simulink model "rfsoc4x2_ospfb_128"  (R2021a)
settings: Solver=VariableStepAuto  StartTime=0.0  StopTime=2048  RelTol=1e-3
undefined symbols (not defined in the file): pfb_coeff_gen_calc
libraries: xbsIndex_r4 x37092, casper_library_delays x737, casper_library_misc x68, xps_library x1
(part 228 of 339)

== system rfsoc4x2_ospfb_128/fft_wideband_real1/fft_direct/butterfly0_0/twiddle/bus_mult ==
  a : Inport
  b : Inport  Port=2
  misci : Inport  Port=3
  a*b_bussify : Subsystem  AncestorBlock=casper_library_flow_control/bus_create  mask(bus_create){inputNum=8}
      mask prompts: inputNum "Number of inputs:"
      mask init:
      | bus_create_init(gcb,...
      |     'inputNum', inputNum);
  a_debus : Subsystem  AncestorBlock=casper_library_flow_control/bus_expand  mask(bus_expand){mode=divisions of arbitrary size, outputNum=2, outputWidth=36, outputBinaryPt=0, outputArithmeticType=0, show_format=on, outputToWorkspace=off, variablePrefix=, outputToModelAsWell=on}
      mask prompts: outputNum "Number of outputs:"; outputWidth "Output width:"; outputBinaryPt "Output binary point position:"; outputArithmeticType "Output arithmetic type (ufix=0, fix=1, bool=2):"; show_format "Print format string?"; outputToWorkspace "Output to workspace?"; variablePrefix "Variable name prefix:"; outputToModelAsWell "Output to model as well?"
      mask help:
      | Expands a 'bus' made using a bus_create or Xilinx
      | concat block.
      | The input will be divided into the specified number
      | of outputs with the specified arithmetic types.
      | Divisions are made from most significant bit.
      mask init: same as rfsoc4x2_ospfb_128/bus_expand1
      settings: AttributesFormatString=1 outputs: uf36.0,
      mask TypeOptions mode: divisions of equal size | divisions of arbitrary size
      mask Callback mode: %bus_expand_callback();
      mask Callback outputWidth: %bus_expand_callback();
      mask Callback outputToWorkspace: %bus_expand_callback();
  b_debus : Subsystem  AncestorBlock=casper_library_flow_control/bus_expand  mask(bus_expand){mode=divisions of arbitrary size, outputNum=2, outputWidth=[36 36 36 36 36 36 36 36], outputBinaryPt=[0 0 0 0 0 0 0 0], outputArithmeticType=[0 0 0 0 0 0 0 0], show_format=on, outputToWorkspace=off, variablePrefix=, outputToModelAsWell=on}
      mask prompts: outputNum "Number of outputs:"; outputWidth "Output width:"; outputBinaryPt "Output binary point position:"; outputArithmeticType "Output arithmetic type (ufix=0, fix=1, bool=2):"; show_format "Print format string?"; outputToWorkspace "Output to workspace?"; variablePrefix "Variable name prefix:"; outputToModelAsWell "Output to model as well?"
      mask help:
      | Expands a 'bus' made using a bus_create or Xilinx
      | concat block.
      | The input will be divided into the specified number
      | of outputs with the specified arithmetic types.
      | Divisions are made from most significant bit.
      mask init: same as rfsoc4x2_ospfb_128/bus_expand1
      settings: AttributesFormatString=8 outputs: uf36.0,uf36.0,uf36.0,uf36.0,uf36.0,uf36.0,uf36.0,uf36.0,
      mask TypeOptions mode: divisions of equal size | divisions of arbitrary size
      mask Callback mode: %bus_expand_callback();
      mask Callback outputWidth: %bus_expand_callback();
      mask Callback outputToWorkspace: %bus_expand_callback();
  dmisc : xbsIndex_r4/Delay  rst=off  infoeditControl=Selection of Reset will increase slice count due to use of real FFs and instead of SRLs  en=off  latency=mult_latency+add_latency+conv_latency+fan_latency  reg_retiming=on  dbl_ovrd=off  block_type=delay
  mult1 : Subsystem  AncestorBlock=casper_library_multipliers/cmult  mask(cmult){n_bits_a=18, bin_pt_a=17, n_bits_b=18, bin_pt_b=17, n_bits_ab=37, bin_pt_ab=34, quantization=Truncate, overflow=Wrap, conjugated=off, async=off, pipelined_enable=on, floating_point=off, float_type=single, exp_width=8, frac_width=24, in_latency=0, mult_latency=3, add_latency=1, conv_latency=0, pipeline_cmult_en=off, pipeline_latency=0, multiplier_implementation=behavioral HDL}
      mask prompts: n_bits_a "Number of Bits 'a'"; bin_pt_a "Binary Point 'a'"; n_bits_b "Number of Bits 'b'"; bin_pt_b "Binary Point 'b'"; n_bits_ab "Number of Bits 'ab'"; bin_pt_ab "Binary Point 'ab'"; conjugated "Conjugate"; async "asynchronous operation"; pipelined_enable "enable pipeline"; floating_point "floating point"; float_type "float type"; exp_width "exponent width"; frac_width "fraction width"; in_latency "Input latency"; mult_latency "Multiplier Latency"; add_latency "Adder Latency"; conv_latency "Convert latency"; pipeline_cmult_en "Pipeline cmult enable"; pipeline_latency "Pipeline latency"; multiplier_implementation "Multiplier implementation"
      mask help:
      | Multiplies two complex numbers using 4 multipliers and 2 adders.
      | Conjugation is optional.
      mask init: same as rfsoc4x2_ospfb_128/fft2/fft_direct/butterfly0_0/twiddle/bus_mult/mult1
      settings: AttributesFormatString=|
      | 18_17 * 18_17 ==> 37_34
      | Truncate, Wrap
      | Latency=0
      mask TypeOptions quantization: Truncate | Round  (unbiased: +/- Inf) | Round  (unbiased: Even Values)
      mask TypeOptions overflow: Wrap | Saturate | Flag as error
      mask Callback floating_point:
      | onoff = get_param(gcb, 'floating_point');
      | if strcmp(onoff,'on')
      |     enable_fixpt = 'off';
      |     set_param_state(gcb, 'float_type', 'on')
      | 
      |     f_type = get_param(gcb, 'float_type');
      |     if strcmp(f_type,'custom')
      |         set_param_state(gcb, 'exp_width', 'on')
      |         set_param_state(gcb, 'frac_width', 'on')
      |     else
      |         set_param_state(gcb, 'exp_width', 'off')
      |         set_param_state(gcb, 'frac_width', 'off')
      |     end
      | 
      | 
      | else
      |     enable_fixpt = 'on';
      |     set_param_state(gcb, 'float_type', 'off')
      |     set_param_state(gcb, 'exp_width', 'off')
      |     set_param_state(gcb, 'frac_width', 'off')
      | end
      | 
      | 
      | set_param_state(gcb, 'n_bits_a', enable_fixpt)
      | set_param_state(gcb, 'bin_pt_a', enable_fixpt)
      | set_param_state(gcb, 'n_bits_b', enable_fixpt)
      | set_param_state(gcb, 'bin_pt_b', enable_fixpt)
      | set_param_state(gcb, 'n_bits_ab', enable_fixpt)
      | set_param_state(gcb, 'bin_pt_ab', enable_fixpt)
      mask TypeOptions float_type: single | custom
      mask Callback float_type:
      | f_type = get_param(gcb, 'float_type');
      | if strcmp(f_type,'custom')
      |     set_param_state(gcb, 'exp_width', 'on')
      |     set_param_state(gcb, 'frac_width', 'on')
      | else
      |     set_param_state(gcb, 'exp_width', 'off')
      |     set_param_state(gcb, 'frac_width', 'off')
      | end
      mask Callback pipeline_cmult_en:
      | pipeline_en = get_param(gcb, 'pipeline_cmult_en');
      | if strcmp(pipeline_en,'on')
      | 
      |     set_param_state(gcb, 'pipeline_latency', 'on')
      | else
      |     set_param_state(gcb, 'pipeline_latency', 'off')
      | end
      mask TypeOptions multiplier_implementation: behavioral HDL | standard core | embedded multiplier core
      mask DialogControl ParameterTabVar0 Prompt: basic
      mask DialogControl ParameterTabVar01 Prompt: latency
      mask DialogControl ParameterTabVar012 Prompt: implementation
  mult2 : Subsystem  AncestorBlock=casper_library_multipliers/cmult  mask(cmult){n_bits_a=18, bin_pt_a=17, n_bits_b=18, bin_pt_b=17, n_bits_ab=37, bin_pt_ab=34, quantization=Truncate, overflow=Wrap, conjugated=off, async=off, pipelined_enable=on, floating_point=off, float_type=single, exp_width=8, frac_width=24, in_latency=0, mult_latency=3, add_latency=1, conv_latency=0, pipeline_cmult_en=off, pipeline_latency=0, multiplier_implementation=behavioral HDL}
      mask prompts: n_bits_a "Number of Bits 'a'"; bin_pt_a "Binary Point 'a'"; n_bits_b "Number of Bits 'b'"; bin_pt_b "Binary Point 'b'"; n_bits_ab "Number of Bits 'ab'"; bin_pt_ab "Binary Point 'ab'"; conjugated "Conjugate"; async "asynchronous operation"; pipelined_enable "enable pipeline"; floating_point "floating point"; float_type "float type"; exp_width "exponent width"; frac_width "fraction width"; in_latency "Input latency"; mult_latency "Multiplier Latency"; add_latency "Adder Latency"; conv_latency "Convert latency"; pipeline_cmult_en "Pipeline cmult enable"; pipeline_latency "Pipeline latency"; multiplier_implementation "Multiplier implementation"
      mask help:
      | Multiplies two complex numbers using 4 multipliers and 2 adders.
      | Conjugation is optional.
      mask init: same as rfsoc4x2_ospfb_128/fft2/fft_direct/butterfly0_0/twiddle/bus_mult/mult1
      settings: AttributesFormatString=|
      | 18_17 * 18_17 ==> 37_34
      | Truncate, Wrap
      | Latency=0
      mask TypeOptions quantization: Truncate | Round  (unbiased: +/- Inf) | Round  (unbiased: Even Values)
      mask TypeOptions overflow: Wrap | Saturate | Flag as error
      mask Callback floating_point:
      | onoff = get_param(gcb, 'floating_point');
      | if strcmp(onoff,'on')
      |     enable_fixpt = 'off';
      |     set_param_state(gcb, 'float_type', 'on')
      | 
      |     f_type = get_param(gcb, 'float_type');
      |     if strcmp(f_type,'custom')
      |         set_param_state(gcb, 'exp_width', 'on')
      |         set_param_state(gcb, 'frac_width', 'on')
      |     else
      |         set_param_state(gcb, 'exp_width', 'off')
      |         set_param_state(gcb, 'frac_width', 'off')
      |     end
      | 
      | 
      | else
      |     enable_fixpt = 'on';
      |     set_param_state(gcb, 'float_type', 'off')
      |     set_param_state(gcb, 'exp_width', 'off')
      |     set_param_state(gcb, 'frac_width', 'off')
      | end
      | 
      | 
      | set_param_state(gcb, 'n_bits_a', enable_fixpt)
      | set_param_state(gcb, 'bin_pt_a', enable_fixpt)
      | set_param_state(gcb, 'n_bits_b', enable_fixpt)
      | set_param_state(gcb, 'bin_pt_b', enable_fixpt)
      | set_param_state(gcb, 'n_bits_ab', enable_fixpt)
      | set_param_state(gcb, 'bin_pt_ab', enable_fixpt)
      mask TypeOptions float_type: single | custom
      mask Callback float_type:
      | f_type = get_param(gcb, 'float_type');
      | if strcmp(f_type,'custom')
      |     set_param_state(gcb, 'exp_width', 'on')
      |     set_param_state(gcb, 'frac_width', 'on')
      | else
      |     set_param_state(gcb, 'exp_width', 'off')
      |     set_param_state(gcb, 'frac_width', 'off')
      | end
      mask Callback pipeline_cmult_en:
      | pipeline_en = get_param(gcb, 'pipeline_cmult_en');
      | if strcmp(pipeline_en,'on')
      | 
      |     set_param_state(gcb, 'pipeline_latency', 'on')
      | else
      |     set_param_state(gcb, 'pipeline_latency', 'off')
      | end
      mask TypeOptions multiplier_implementation: behavioral HDL | standard core | embedded multiplier core
      mask DialogControl ParameterTabVar0 Prompt: basic
      mask DialogControl ParameterTabVar01 Prompt: latency
      mask DialogControl ParameterTabVar012 Prompt: implementation
  mult3 : Subsystem  AncestorBlock=casper_library_multipliers/cmult  mask(cmult){n_bits_a=18, bin_pt_a=17, n_bits_b=18, bin_pt_b=17, n_bits_ab=37, bin_pt_ab=34, quantization=Truncate, overflow=Wrap, conjugated=off, async=off, pipelined_enable=on, floating_point=off, float_type=single, exp_width=8, frac_width=24, in_latency=0, mult_latency=3, add_latency=1, conv_latency=0, pipeline_cmult_en=off, pipeline_latency=0, multiplier_implementation=behavioral HDL}
      mask prompts: n_bits_a "Number of Bits 'a'"; bin_pt_a "Binary Point 'a'"; n_bits_b "Number of Bits 'b'"; bin_pt_b "Binary Point 'b'"; n_bits_ab "Number of Bits 'ab'"; bin_pt_ab "Binary Point 'ab'"; conjugated "Conjugate"; async "asynchronous operation"; pipelined_enable "enable pipeline"; floating_point "floating point"; float_type "float type"; exp_width "exponent width"; frac_width "fraction width"; in_latency "Input latency"; mult_latency "Multiplier Latency"; add_latency "Adder Latency"; conv_latency "Convert latency"; pipeline_cmult_en "Pipeline cmult enable"; pipeline_latency "Pipeline latency"; multiplier_implementation "Multiplier implementation"
      mask help:
      | Multiplies two complex numbers using 4 multipliers and 2 adders.
      | Conjugation is optional.
      mask init: same as rfsoc4x2_ospfb_128/fft2/fft_direct/butterfly0_0/twiddle/bus_mult/mult1
      settings: AttributesFormatString=|
      | 18_17 * 18_17 ==> 37_34
      | Truncate, Wrap
      | Latency=0
      mask TypeOptions quantization: Truncate | Round  (unbiased: +/- Inf) | Round  (unbiased: Even Values)
      mask TypeOptions overflow: Wrap | Saturate | Flag as error
      mask Callback floating_point:
      | onoff = get_param(gcb, 'floating_point');
      | if strcmp(onoff,'on')
      |     enable_fixpt = 'off';
      |     set_param_state(gcb, 'float_type', 'on')
      | 
      |     f_type = get_param(gcb, 'float_type');
      |     if strcmp(f_type,'custom')
      |         set_param_state(gcb, 'exp_width', 'on')
      |         set_param_state(gcb, 'frac_width', 'on')
      |     else
      |         set_param_state(gcb, 'exp_width', 'off')
      |         set_param_state(gcb, 'frac_width', 'off')
      |     end
      | 
      | 
      | else
      |     enable_fixpt = 'on';
      |     set_param_state(gcb, 'float_type', 'off')
      |     set_param_state(gcb, 'exp_width', 'off')
      |     set_param_state(gcb, 'frac_width', 'off')
      | end
      | 
      | 
      | set_param_state(gcb, 'n_bits_a', enable_fixpt)
      | set_param_state(gcb, 'bin_pt_a', enable_fixpt)
      | set_param_state(gcb, 'n_bits_b', enable_fixpt)
      | set_param_state(gcb, 'bin_pt_b', enable_fixpt)
      | set_param_state(gcb, 'n_bits_ab', enable_fixpt)
      | set_param_state(gcb, 'bin_pt_ab', enable_fixpt)
      mask TypeOptions float_type: single | custom
      mask Callback float_type:
      | f_type = get_param(gcb, 'float_type');
      | if strcmp(f_type,'custom')
      |     set_param_state(gcb, 'exp_width', 'on')
      |     set_param_state(gcb, 'frac_width', 'on')
      | else
      |     set_param_state(gcb, 'exp_width', 'off')
      |     set_param_state(gcb, 'frac_width', 'off')
      | end
      mask Callback pipeline_cmult_en:
      | pipeline_en = get_param(gcb, 'pipeline_cmult_en');
      | if strcmp(pipeline_en,'on')
      | 
      |     set_param_state(gcb, 'pipeline_latency', 'on')
      | else
      |     set_param_state(gcb, 'pipeline_latency', 'off')
      | end
      mask TypeOptions multiplier_implementation: behavioral HDL | standard core | embedded multiplier core
      mask DialogControl ParameterTabVar0 Prompt: basic
      mask DialogControl ParameterTabVar01 Prompt: latency
      mask DialogControl ParameterTabVar012 Prompt: implementation
  mult4 : Subsystem  AncestorBlock=casper_library_multipliers/cmult  mask(cmult){n_bits_a=18, bin_pt_a=17, n_bits_b=18, bin_pt_b=17, n_bits_ab=37, bin_pt_ab=34, quantization=Truncate, overflow=Wrap, conjugated=off, async=off, pipelined_enable=on, floating_point=off, float_type=single, exp_width=8, frac_width=24, in_latency=0, mult_latency=3, add_latency=1, conv_latency=0, pipeline_cmult_en=off, pipeline_latency=0, multiplier_implementation=behavioral HDL}
      mask prompts: n_bits_a "Number of Bits 'a'"; bin_pt_a "Binary Point 'a'"; n_bits_b "Number of Bits 'b'"; bin_pt_b "Binary Point 'b'"; n_bits_ab "Number of Bits 'ab'"; bin_pt_ab "Binary Point 'ab'"; conjugated "Conjugate"; async "asynchronous operation"; pipelined_enable "enable pipeline"; floating_point "floating point"; float_type "float type"; exp_width "exponent width"; frac_width "fraction width"; in_latency "Input latency"; mult_latency "Multiplier Latency"; add_latency "Adder Latency"; conv_latency "Convert latency"; pipeline_cmult_en "Pipeline cmult enable"; pipeline_latency "Pipeline latency"; multiplier_implementation "Multiplier implementation"
      mask help:
      | Multiplies two complex numbers using 4 multipliers and 2 adders.
      | Conjugation is optional.
      mask init: same as rfsoc4x2_ospfb_128/fft2/fft_direct/butterfly0_0/twiddle/bus_mult/mult1
      settings: AttributesFormatString=|
      | 18_17 * 18_17 ==> 37_34
      | Truncate, Wrap
      | Latency=0
      mask TypeOptions quantization: Truncate | Round  (unbiased: +/- Inf) | Round  (unbiased: Even Values)
      mask TypeOptions overflow: Wrap | Saturate | Flag as error
      mask Callback floating_point:
      | onoff = get_param(gcb, 'floating_point');
      | if strcmp(onoff,'on')
      |     enable_fixpt = 'off';
      |     set_param_state(gcb, 'float_type', 'on')
      | 
      |     f_type = get_param(gcb, 'float_type');
      |     if strcmp(f_type,'custom')
      |         set_param_state(gcb, 'exp_width', 'on')
      |         set_param_state(gcb, 'frac_width', 'on')
      |     else
      |         set_param_state(gcb, 'exp_width', 'off')
      |         set_param_state(gcb, 'frac_width', 'off')
      |     end
      | 
      | 
      | else
      |     enable_fixpt = 'on';
      |     set_param_state(gcb, 'float_type', 'off')
      |     set_param_state(gcb, 'exp_width', 'off')
      |     set_param_state(gcb, 'frac_width', 'off')
      | end
      | 
      | 
      | set_param_state(gcb, 'n_bits_a', enable_fixpt)
      | set_param_state(gcb, 'bin_pt_a', enable_fixpt)
      | set_param_state(gcb, 'n_bits_b', enable_fixpt)
      | set_param_state(gcb, 'bin_pt_b', enable_fixpt)
      | set_param_state(gcb, 'n_bits_ab', enable_fixpt)
      | set_param_state(gcb, 'bin_pt_ab', enable_fixpt)
      mask TypeOptions float_type: single | custom
      mask Callback float_type:
      | f_type = get_param(gcb, 'float_type');
      | if strcmp(f_type,'custom')
      |     set_param_state(gcb, 'exp_width', 'on')
      |     set_param_state(gcb, 'frac_width', 'on')
      | else
      |     set_param_state(gcb, 'exp_width', 'off')
      |     set_param_state(gcb, 'frac_width', 'off')
      | end
      mask Callback pipeline_cmult_en:
      | pipeline_en = get_param(gcb, 'pipeline_cmult_en');
      | if strcmp(pipeline_en,'on')
      | 
      |     set_param_state(gcb, 'pipeline_latency', 'on')
      | else
      |     set_param_state(gcb, 'pipeline_latency', 'off')
      | end
      mask TypeOptions multiplier_implementation: behavioral HDL | standard core | embedded multiplier core
      mask DialogControl ParameterTabVar0 Prompt: basic
      mask DialogControl ParameterTabVar01 Prompt: latency
      mask DialogControl ParameterTabVar012 Prompt: implementation
  mult5 : Subsystem  AncestorBlock=casper_library_multipliers/cmult  mask(cmult){n_bits_a=18, bin_pt_a=17, n_bits_b=18, bin_pt_b=17, n_bits_ab=37, bin_pt_ab=34, quantization=Truncate, overflow=Wrap, conjugated=off, async=off, pipelined_enable=on, floating_point=off, float_type=single, exp_width=8, frac_width=24, in_latency=0, mult_latency=3, add_latency=1, conv_latency=0, pipeline_cmult_en=off, pipeline_latency=0, multiplier_implementation=behavioral HDL}
      mask prompts: n_bits_a "Number of Bits 'a'"; bin_pt_a "Binary Point 'a'"; n_bits_b "Number of Bits 'b'"; bin_pt_b "Binary Point 'b'"; n_bits_ab "Number of Bits 'ab'"; bin_pt_ab "Binary Point 'ab'"; conjugated "Conjugate"; async "asynchronous operation"; pipelined_enable "enable pipeline"; floating_point "floating point"; float_type "float type"; exp_width "exponent width"; frac_width "fraction width"; in_latency "Input latency"; mult_latency "Multiplier Latency"; add_latency "Adder Latency"; conv_latency "Convert latency"; pipeline_cmult_en "Pipeline cmult enable"; pipeline_latency "Pipeline latency"; multiplier_implementation "Multiplier implementation"
      mask help:
      | Multiplies two complex numbers using 4 multipliers and 2 adders.
      | Conjugation is optional.
      mask init: same as rfsoc4x2_ospfb_128/fft2/fft_direct/butterfly0_0/twiddle/bus_mult/mult1
      settings: AttributesFormatString=|
      | 18_17 * 18_17 ==> 37_34
      | Truncate, Wrap
      | Latency=0
      mask TypeOptions quantization: Truncate | Round  (unbiased: +/- Inf) | Round  (unbiased: Even Values)
      mask TypeOptions overflow: Wrap | Saturate | Flag as error
      mask Callback floating_point:
      | onoff = get_param(gcb, 'floating_point');
      | if strcmp(onoff,'on')
      |     enable_fixpt = 'off';
      |     set_param_state(gcb, 'float_type', 'on')
      | 
      |     f_type = get_param(gcb, 'float_type');
      |     if strcmp(f_type,'custom')
      |         set_param_state(gcb, 'exp_width', 'on')
      |         set_param_state(gcb, 'frac_width', 'on')
      |     else
      |         set_param_state(gcb, 'exp_width', 'off')
      |         set_param_state(gcb, 'frac_width', 'off')
      |     end
      | 
      | 
      | else
      |     enable_fixpt = 'on';
      |     set_param_state(gcb, 'float_type', 'off')
      |     set_param_state(gcb, 'exp_width', 'off')
      |     set_param_state(gcb, 'frac_width', 'off')
      | end
      | 
      | 
      | set_param_state(gcb, 'n_bits_a', enable_fixpt)
      | set_param_state(gcb, 'bin_pt_a', enable_fixpt)
      | set_param_state(gcb, 'n_bits_b', enable_fixpt)
      | set_param_state(gcb, 'bin_pt_b', enable_fixpt)
      | set_param_state(gcb, 'n_bits_ab', enable_fixpt)
      | set_param_state(gcb, 'bin_pt_ab', enable_fixpt)
      mask TypeOptions float_type: single | custom
      mask Callback float_type:
      | f_type = get_param(gcb, 'float_type');
      | if strcmp(f_type,'custom')
      |     set_param_state(gcb, 'exp_width', 'on')
      |     set_param_state(gcb, 'frac_width', 'on')
      | else
      |     set_param_state(gcb, 'exp_width', 'off')
      |     set_param_state(gcb, 'frac_width', 'off')
      | end
      mask Callback pipeline_cmult_en:
      | pipeline_en = get_param(gcb, 'pipeline_cmult_en');
      | if strcmp(pipeline_en,'on')
      | 
      |     set_param_state(gcb, 'pipeline_latency', 'on')
      | else
      |     set_param_state(gcb, 'pipeline_latency', 'off')
      | end
      mask TypeOptions multiplier_implementation: behavioral HDL | standard core | embedded multiplier core
      mask DialogControl ParameterTabVar0 Prompt: basic
      mask DialogControl ParameterTabVar01 Prompt: latency
      mask DialogControl ParameterTabVar012 Prompt: implementation
  mult6 : Subsystem  AncestorBlock=casper_library_multipliers/cmult  mask(cmult){n_bits_a=18, bin_pt_a=17, n_bits_b=18, bin_pt_b=17, n_bits_ab=37, bin_pt_ab=34, quantization=Truncate, overflow=Wrap, conjugated=off, async=off, pipelined_enable=on, floating_point=off, float_type=single, exp_width=8, frac_width=24, in_latency=0, mult_latency=3, add_latency=1, conv_latency=0, pipeline_cmult_en=off, pipeline_latency=0, multiplier_implementation=behavioral HDL}
      mask prompts: n_bits_a "Number of Bits 'a'"; bin_pt_a "Binary Point 'a'"; n_bits_b "Number of Bits 'b'"; bin_pt_b "Binary Point 'b'"; n_bits_ab "Number of Bits 'ab'"; bin_pt_ab "Binary Point 'ab'"; conjugated "Conjugate"; async "asynchronous operation"; pipelined_enable "enable pipeline"; floating_point "floating point"; float_type "float type"; exp_width "exponent width"; frac_width "fraction width"; in_latency "Input latency"; mult_latency "Multiplier Latency"; add_latency "Adder Latency"; conv_latency "Convert latency"; pipeline_cmult_en "Pipeline cmult enable"; pipeline_latency "Pipeline latency"; multiplier_implementation "Multiplier implementation"
      mask help:
      | Multiplies two complex numbers using 4 multipliers and 2 adders.
      | Conjugation is optional.
      mask init: same as rfsoc4x2_ospfb_128/fft2/fft_direct/butterfly0_0/twiddle/bus_mult/mult1
      settings: AttributesFormatString=|
      | 18_17 * 18_17 ==> 37_34
      | Truncate, Wrap
      | Latency=0
      mask TypeOptions quantization: Truncate | Round  (unbiased: +/- Inf) | Round  (unbiased: Even Values)
      mask TypeOptions overflow: Wrap | Saturate | Flag as error
      mask Callback floating_point:
      | onoff = get_param(gcb, 'floating_point');
      | if strcmp(onoff,'on')
      |     enable_fixpt = 'off';
      |     set_param_state(gcb, 'float_type', 'on')
      | 
      |     f_type = get_param(gcb, 'float_type');
      |     if strcmp(f_type,'custom')
      |         set_param_state(gcb, 'exp_width', 'on')
      |         set_param_state(gcb, 'frac_width', 'on')
      |     else
      |         set_param_state(gcb, 'exp_width', 'off')
      |         set_param_state(gcb, 'frac_width', 'off')
      |     end
      | 
      | 
      | else
      |     enable_fixpt = 'on';
      |     set_param_state(gcb, 'float_type', 'off')
      |     set_param_state(gcb, 'exp_width', 'off')
      |     set_param_state(gcb, 'frac_width', 'off')
      | end
      | 
      | 
      | set_param_state(gcb, 'n_bits_a', enable_fixpt)
      | set_param_state(gcb, 'bin_pt_a', enable_fixpt)
      | set_param_state(gcb, 'n_bits_b', enable_fixpt)
      | set_param_state(gcb, 'bin_pt_b', enable_fixpt)
      | set_param_state(gcb, 'n_bits_ab', enable_fixpt)
      | set_param_state(gcb, 'bin_pt_ab', enable_fixpt)
      mask TypeOptions float_type: single | custom
      mask Callback float_type:
      | f_type = get_param(gcb, 'float_type');
      | if strcmp(f_type,'custom')
      |     set_param_state(gcb, 'exp_width', 'on')
      |     set_param_state(gcb, 'frac_width', 'on')
      | else
      |     set_param_state(gcb, 'exp_width', 'off')
      |     set_param_state(gcb, 'frac_width', 'off')
      | end
      mask Callback pipeline_cmult_en:
      | pipeline_en = get_param(gcb, 'pipeline_cmult_en');
      | if strcmp(pipeline_en,'on')
      | 
      |     set_param_state(gcb, 'pipeline_latency', 'on')
      | else
      |     set_param_state(gcb, 'pipeline_latency', 'off')
      | end
      mask TypeOptions multiplier_implementation: behavioral HDL | standard core | embedded multiplier core
      mask DialogControl ParameterTabVar0 Prompt: basic
      mask DialogControl ParameterTabVar01 Prompt: latency
      mask DialogControl ParameterTabVar012 Prompt: implementation
  mult7 : Subsystem  AncestorBlock=casper_library_multipliers/cmult  mask(cmult){n_bits_a=18, bin_pt_a=17, n_bits_b=18, bin_pt_b=17, n_bits_ab=37, bin_pt_ab=34, quantization=Truncate, overflow=Wrap, conjugated=off, async=off, pipelined_enable=on, floating_point=off, float_type=single, exp_width=8, frac_width=24, in_latency=0, mult_latency=3, add_latency=1, conv_latency=0, pipeline_cmult_en=off, pipeline_latency=0, multiplier_implementation=behavioral HDL}
      mask prompts: n_bits_a "Number of Bits 'a'"; bin_pt_a "Binary Point 'a'"; n_bits_b "Number of Bits 'b'"; bin_pt_b "Binary Point 'b'"; n_bits_ab "Number of Bits 'ab'"; bin_pt_ab "Binary Point 'ab'"; conjugated "Conjugate"; async "asynchronous operation"; pipelined_enable "enable pipeline"; floating_point "floating point"; float_type "float type"; exp_width "exponent width"; frac_width "fraction width"; in_latency "Input latency"; mult_latency "Multiplier Latency"; add_latency "Adder Latency"; conv_latency "Convert latency"; pipeline_cmult_en "Pipeline cmult enable"; pipeline_latency "Pipeline latency"; multiplier_implementation "Multiplier implementation"
      mask help:
      | Multiplies two complex numbers using 4 multipliers and 2 adders.
      | Conjugation is optional.
      mask init: same as rfsoc4x2_ospfb_128/fft2/fft_direct/butterfly0_0/twiddle/bus_mult/mult1
      settings: AttributesFormatString=|
      | 18_17 * 18_17 ==> 37_34
      | Truncate, Wrap
      | Latency=0
      mask TypeOptions quantization: Truncate | Round  (unbiased: +/- Inf) | Round  (unbiased: Even Values)
      mask TypeOptions overflow: Wrap | Saturate | Flag as error
      mask Callback floating_point:
      | onoff = get_param(gcb, 'floating_point');
      | if strcmp(onoff,'on')
      |     enable_fixpt = 'off';
      |     set_param_state(gcb, 'float_type', 'on')
      | 
      |     f_type = get_param(gcb, 'float_type');
      |     if strcmp(f_type,'custom')
      |         set_param_state(gcb, 'exp_width', 'on')
      |         set_param_state(gcb, 'frac_width', 'on')
      |     else
      |         set_param_state(gcb, 'exp_width', 'off')
      |         set_param_state(gcb, 'frac_width', 'off')
      |     end
      | 
      | 
      | else
      |     enable_fixpt = 'on';
      |     set_param_state(gcb, 'float_type', 'off')
      |     set_param_state(gcb, 'exp_width', 'off')
      |     set_param_state(gcb, 'frac_width', 'off')
      | end
      | 
      | 
      | set_param_state(gcb, 'n_bits_a', enable_fixpt)
      | set_param_state(gcb, 'bin_pt_a', enable_fixpt)
      | set_param_state(gcb, 'n_bits_b', enable_fixpt)
      | set_param_state(gcb, 'bin_pt_b', enable_fixpt)
      | set_param_state(gcb, 'n_bits_ab', enable_fixpt)
      | set_param_state(gcb, 'bin_pt_ab', enable_fixpt)
      mask TypeOptions float_type: single | custom
      mask Callback float_type:
      | f_type = get_param(gcb, 'float_type');
      | if strcmp(f_type,'custom')
      |     set_param_state(gcb, 'exp_width', 'on')
      |     set_param_state(gcb, 'frac_width', 'on')
      | else
      |     set_param_state(gcb, 'exp_width', 'off')
      |     set_param_state(gcb, 'frac_width', 'off')
      | end
      mask Callback pipeline_cmult_en:
      | pipeline_en = get_param(gcb, 'pipeline_cmult_en');
      | if strcmp(pipeline_en,'on')
      | 
      |     set_param_state(gcb, 'pipeline_latency', 'on')
      | else
      |     set_param_state(gcb, 'pipeline_latency', 'off')
      | end
      mask TypeOptions multiplier_implementation: behavioral HDL | standard core | embedded multiplier core
      mask DialogControl ParameterTabVar0 Prompt: basic
      mask DialogControl ParameterTabVar01 Prompt: latency
      mask DialogControl ParameterTabVar012 Prompt: implementation
  mult8 : Subsystem  AncestorBlock=casper_library_multipliers/cmult  mask(cmult){n_bits_a=18, bin_pt_a=17, n_bits_b=18, bin_pt_b=17, n_bits_ab=37, bin_pt_ab=34, quantization=Truncate, overflow=Wrap, conjugated=off, async=off, pipelined_enable=on, floating_point=off, float_type=single, exp_width=8, frac_width=24, in_latency=0, mult_latency=3, add_latency=1, conv_latency=0, pipeline_cmult_en=off, pipeline_latency=0, multiplier_implementation=behavioral HDL}
      mask prompts: n_bits_a "Number of Bits 'a'"; bin_pt_a "Binary Point 'a'"; n_bits_b "Number of Bits 'b'"; bin_pt_b "Binary Point 'b'"; n_bits_ab "Number of Bits 'ab'"; bin_pt_ab "Binary Point 'ab'"; conjugated "Conjugate"; async "asynchronous operation"; pipelined_enable "enable pipeline"; floating_point "floating point"; float_type "float type"; exp_width "exponent width"; frac_width "fraction width"; in_latency "Input latency"; mult_latency "Multiplier Latency"; add_latency "Adder Latency"; conv_latency "Convert latency"; pipeline_cmult_en "Pipeline cmult enable"; pipeline_latency "Pipeline latency"; multiplier_implementation "Multiplier implementation"
      mask help:
      | Multiplies two complex numbers using 4 multipliers and 2 adders.
      | Conjugation is optional.
      mask init: same as rfsoc4x2_ospfb_128/fft2/fft_direct/butterfly0_0/twiddle/bus_mult/mult1
      settings: AttributesFormatString=|
      | 18_17 * 18_17 ==> 37_34
      | Truncate, Wrap
      | Latency=0
      mask TypeOptions quantization: Truncate | Round  (unbiased: +/- Inf) | Round  (unbiased: Even Values)
      mask TypeOptions overflow: Wrap | Saturate | Flag as error
      mask Callback floating_point:
      | onoff = get_param(gcb, 'floating_point');
      | if strcmp(onoff,'on')
      |     enable_fixpt = 'off';
      |     set_param_state(gcb, 'float_type', 'on')
      | 
      |     f_type = get_param(gcb, 'float_type');
      |     if strcmp(f_type,'custom')
      |         set_param_state(gcb, 'exp_width', 'on')
      |         set_param_state(gcb, 'frac_width', 'on')
      |     else
      |         set_param_state(gcb, 'exp_width', 'off')
      |         set_param_state(gcb, 'frac_width', 'off')
      |     end
      | 
      | 
      | else
      |     enable_fixpt = 'on';
      |     set_param_state(gcb, 'float_type', 'off')
      |     set_param_state(gcb, 'exp_width', 'off')
      |     set_param_state(gcb, 'frac_width', 'off')
      | end
      | 
      | 
      | set_param_state(gcb, 'n_bits_a', enable_fixpt)
      | set_param_state(gcb, 'bin_pt_a', enable_fixpt)
      | set_param_state(gcb, 'n_bits_b', enable_fixpt)
      | set_param_state(gcb, 'bin_pt_b', enable_fixpt)
      | set_param_state(gcb, 'n_bits_ab', enable_fixpt)
      | set_param_state(gcb, 'bin_pt_ab', enable_fixpt)
      mask TypeOptions float_type: single | custom
      mask Callback float_type:
      | f_type = get_param(gcb, 'float_type');
      | if strcmp(f_type,'custom')
      |     set_param_state(gcb, 'exp_width', 'on')
      |     set_param_state(gcb, 'frac_width', 'on')
      | else
      |     set_param_state(gcb, 'exp_width', 'off')
      |     set_param_state(gcb, 'frac_width', 'off')
      | end
      mask Callback pipeline_cmult_en:
      | pipeline_en = get_param(gcb, 'pipeline_cmult_en');
      | if strcmp(pipeline_en,'on')
      | 
      |     set_param_state(gcb, 'pipeline_latency', 'on')
      | else
      |     set_param_state(gcb, 'pipeline_latency', 'off')
      | end
      mask TypeOptions multiplier_implementation: behavioral HDL | standard core | embedded multiplier core
      mask DialogControl ParameterTabVar0 Prompt: basic
      mask DialogControl ParameterTabVar01 Prompt: latency
      mask DialogControl ParameterTabVar012 Prompt: implementation
  repa : Subsystem  AncestorBlock=casper_library_bus/bus_replicate  mask(bus_replicate){replication=1, csp_latency=0, misc=off, implementation=core}
      mask prompts: replication "replication factor"; csp_latency "latency"; misc "misc support"; implementation "delay implementation"
      mask help: Output bus formed by replicating input bus a number of times
      mask init:
      | bus_replicate_init(gcb, ...
      |     'replication', replication, ...
      |     'csp_latency', csp_latency, ...
      |     'implementation', implementation, ...
      |     'misc', misc);
      mask TypeOptions implementation: core | behavioral
  repb : Subsystem  AncestorBlock=casper_library_bus/bus_replicate  mask(bus_replicate){replication=1, csp_latency=0, misc=off, implementation=core}
      mask prompts: replication "replication factor"; csp_latency "latency"; misc "misc support"; implementation "delay implementation"
      mask help: Output bus formed by replicating input bus a number of times
      mask init:
      | bus_replicate_init(gcb, ...
      |     'replication', replication, ...
      |     'csp_latency', csp_latency, ...
      |     'implementation', implementation, ...
      |     'misc', misc);
      mask TypeOptions implementation: core | behavioral
  a*b : Outport
  misco : Outport  Port=2
  wires:
  dmisc/1 -> misco/1
  a*b_bussify/1(bus_out) -> a*b/1
  mult8/1(ab) -> a*b_bussify/8(in8)
  mult7/1(ab) -> a*b_bussify/7(in7)
  mult6/1(ab) -> a*b_bussify/6(in6)
  mult5/1(ab) -> a*b_bussify/5(in5)
  mult4/1(ab) -> a*b_bussify/4(in4)
  mult3/1(ab) -> a*b_bussify/3(in3)
  mult2/1(ab) -> a*b_bussify/2(in2)
  mult1/1(ab) -> a*b_bussify/1(in1)
  misci/1 -> dmisc/1
  b_debus/8(lsb_out1) -> mult8/2(b)
  b_debus/7(out2) -> mult7/2(b)
  b_debus/6(out3) -> mult6/2(b)
  b_debus/5(out4) -> mult5/2(b)
  b_debus/4(out5) -> mult4/2(b)
  b_debus/3(out6) -> mult3/2(b)
  b_debus/2(out7) -> mult2/2(b)
  b_debus/1(msb_out8) -> mult1/2(b)
  a_debus/1(msb_lsb_out1) -> mult8/1(a), mult7/1(a), mult6/1(a), mult5/1(a), mult4/1(a), mult3/1(a), mult2/1(a), mult1/1(a)
  repb/1(out) -> b_debus/1(bus_in)
  repa/1(out) -> a_debus/1(bus_in)
  b/1 -> repb/1(in)
  a/1 -> repa/1(in)

== system rfsoc4x2_ospfb_128/fft_wideband_real1/fft_direct/butterfly0_0/twiddle/coeff_gen ==
  rst : Inport
  misci : Inport  Port=2
  Counter : xbsIndex_r4/Counter  cnt_type=Free Running  cnt_to=Inf  operation=Up  start_count=0  cnt_by_val=1  arith_type=Unsigned  n_bits=4  bin_pt=0  load_pin=off  rst=on  en=off  explicit_period=on  period=1  use_behavioral_HDL=on  implementation=Fabric  dbl_ovrd=off  block_type=counter
  Slice : xbsIndex_r4/Slice  nbits=4  boolean_output=off  mode=Upper Bit Location + Width  bit1=0  base1=MSB of Input  bit0=0  base0=LSB of Input  dbl_ovrd=off  block_type=slice
  cosin : Subsystem  Tag=casper:cosin  AncestorBlock=casper_library_downconverter/cosin  mask(cosin){output0=cos, output1=-sin, indep_theta=off, phase=0, fraction=1, table_bits=4, n_bits=18, bin_pt=17, floating_point=off, float_type=single, exp_width=8, frac_width=24, store=1, pack=on, bram=BRAM, misc=on, bram_latency=3, add_latency=1, mux_latency=1, neg_latency=0, conv_latency=3}
      mask prompts: output0 "first output function"; output1 "second output function"; indep_theta "Independent theta values"; phase "initial phase offset (?*(2*pi))"; fraction "fraction of cycle period to output (1/2^?)"; table_bits "samples in cycle period fraction to output (2^?)"; n_bits "bit width"; bin_pt "binary point"; floating_point "floating point"; float_type "float type"; exp_width "exponent width"; frac_width "fraction width"; store "fraction of cycle period to store (1/2^?)"; pack "pack lookup values in same output word"; bram "BRAM implementation"; misc "Miscellaneous port"; bram_latency "bram latency"; add_latency "large adder latency"; mux_latency "mux latency"; neg_latency "negate latency"; conv_latency "convert latency"
      mask init: same as rfsoc4x2_ospfb_128/fft2/fft_direct/butterfly0_0/twiddle/coeff_gen/cosin
      mask TypeOptions output0: sin | cos | -sin | -cos
      mask TypeOptions output1: none | sin | cos | -sin | -cos
      mask Callback floating_point:
      | onoff = get_param(gcb, 'floating_point');
      | if strcmp(onoff,'on')
      |     enable_fixpt = 'off';
      |     set_param_state(gcb, 'float_type', 'on')
      | 
      |     f_type = get_param(gcb, 'float_type');
      |     if strcmp(f_type,'custom')
      |         set_param_state(gcb, 'exp_width', 'on')
      |         set_param_state(gcb, 'frac_width', 'on')
      |     else
      |         set_param_state(gcb, 'exp_width', 'off')
      |         set_param_state(gcb, 'frac_width', 'off')
      |     end
      | 
      | 
      | else
      |     enable_fixpt = 'on';
      |     set_param_state(gcb, 'float_type', 'off')
      |     set_param_state(gcb, 'exp_width', 'off')
      |     set_param_state(gcb, 'frac_width', 'off')
      | end
      | 
      | set_param_state(gcb, 'n_bits', enable_fixpt)
      | set_param_state(gcb, 'bin_pt', enable_fixpt)
      mask TypeOptions float_type: single | custom
      mask Callback float_type:
      | f_type = get_param(gcb, 'float_type');
      | if strcmp(f_type,'custom')
      |     set_param_state(gcb, 'exp_width', 'on')
      |     set_param_state(gcb, 'frac_width', 'on')
      | else
      |     set_param_state(gcb, 'exp_width', 'off')
      |     set_param_state(gcb, 'frac_width', 'off')
      | end
      mask TypeOptions bram: distributed RAM | BRAM
      mask Display:
      | if ~(table_bits == 0),
      |         color('black');port_label('output',1,output0);
      |     color('black');port_label('output',2,output1);
      |     color('black');disp(['z^{-',num2str(add_latency+mux_latency+conv_latency+bram_latency+neg_latency+mux_latency),'}'],'texmode','on');color('black');port_label('input',1,'theta');
      |     if strcmp(misc, 'on'),
      |         color('black');port_label('input',2,'misci');
      |         color('black');port_label('output',3,'misco');
      |     end
      | end
  ri_to_c : casper_library_misc/ri_to_c
      settings: SourceProductName=CASPER DSP Blockset
  w : Outport
  misco : Outport  Port=2
  wires:
  cosin/3(misco) -> misco/1
  misci/1 -> cosin/2(misci)
  cosin/2(-sin) -> ri_to_c/2
  cosin/1(cos) -> ri_to_c/1
  Slice/1 -> cosin/1(theta)
  Counter/1 -> Slice/1
  rst/1 -> Counter/1
  ri_to_c/1 -> w/1

== system rfsoc4x2_ospfb_128/fft_wideband_real1/fft_direct/butterfly1_0/bus_add/a_debus ==
  bus_in : Inport
  reinterpret{1..8} (8 alike) : xbsIndex_r4/Reinterpret  force_arith_type=on  arith_type="Signed  (2's comp)"  force_bin_pt=on  bin_pt=17  block_type=reinterpret
  slice1 : xbsIndex_r4/Slice  nbits=18  boolean_output=off  mode=Upper Bit Location + Width  bit1=-126  base1=MSB of Input  bit0=0  base0=LSB of Input  dbl_ovrd=off  block_type=slice
  slice2 : xbsIndex_r4/Slice  nbits=18  boolean_output=off  mode=Upper Bit Location + Width  bit1=-108  base1=MSB of Input  bit0=0  base0=LSB of Input  dbl_ovrd=off  block_type=slice
  slice3 : xbsIndex_r4/Slice  nbits=18  boolean_output=off  mode=Upper Bit Location + Width  bit1=-90  base1=MSB of Input  bit0=0  base0=LSB of Input  dbl_ovrd=off  block_type=slice
  slice4 : xbsIndex_r4/Slice  nbits=18  boolean_output=off  mode=Upper Bit Location + Width  bit1=-72  base1=MSB of Input  bit0=0  base0=LSB of Input  dbl_ovrd=off  block_type=slice
  slice5 : xbsIndex_r4/Slice  nbits=18  boolean_output=off  mode=Upper Bit Location + Width  bit1=-54  base1=MSB of Input  bit0=0  base0=LSB of Input  dbl_ovrd=off  block_type=slice
  slice6 : xbsIndex_r4/Slice  nbits=18  boolean_output=off  mode=Upper Bit Location + Width  bit1=-36  base1=MSB of Input  bit0=0  base0=LSB of Input  dbl_ovrd=off  block_type=slice
  slice7 : xbsIndex_r4/Slice  nbits=18  boolean_output=off  mode=Upper Bit Location + Width  bit1=-18  base1=MSB of Input  bit0=0  base0=LSB of Input  dbl_ovrd=off  block_type=slice
  slice8 : xbsIndex_r4/Slice  nbits=18  boolean_output=off  mode=Upper Bit Location + Width  bit1=0  base1=MSB of Input  bit0=0  base0=LSB of Input  dbl_ovrd=off  block_type=slice
  msb_out8 : Outport
  out7 : Outport  Port=2
  out6 : Outport  Port=3
  out5 : Outport  Port=4
  out4 : Outport  Port=5
  out3 : Outport  Port=6
  out2 : Outport  Port=7
  lsb_out1 : Outport  Port=8  VectorParamsAs1DForOutWhenUnconnected=off
  wires:
  reinterpret1/1 -> lsb_out1/1
  slice1/1 -> reinterpret1/1
  reinterpret2/1 -> out2/1
  slice2/1 -> reinterpret2/1
  reinterpret3/1 -> out3/1
  slice3/1 -> reinterpret3/1
  reinterpret4/1 -> out4/1
  slice4/1 -> reinterpret4/1
  reinterpret5/1 -> out5/1
  slice5/1 -> reinterpret5/1
  reinterpret6/1 -> out6/1
  slice6/1 -> reinterpret6/1
  reinterpret7/1 -> out7/1
  slice7/1 -> reinterpret7/1
  reinterpret8/1 -> msb_out8/1
  slice8/1 -> reinterpret8/1
  bus_in/1 -> slice1/1, slice2/1, slice3/1, slice4/1, slice5/1, slice6/1, slice7/1, slice8/1

== system rfsoc4x2_ospfb_128/fft_wideband_real1/fft_direct/butterfly1_0/bus_add/b_debus ==
  bus_in : Inport
  reinterpret{1..8} (8 alike) : xbsIndex_r4/Reinterpret  force_arith_type=on  arith_type="Signed  (2's comp)"  force_bin_pt=on  bin_pt=17  block_type=reinterpret
  slice1 : xbsIndex_r4/Slice  nbits=19  boolean_output=off  mode=Upper Bit Location + Width  bit1=-133  base1=MSB of Input  bit0=0  base0=LSB of Input  dbl_ovrd=off  block_type=slice
  slice2 : xbsIndex_r4/Slice  nbits=19  boolean_output=off  mode=Upper Bit Location + Width  bit1=-114  base1=MSB of Input  bit0=0  base0=LSB of Input  dbl_ovrd=off  block_type=slice
  slice3 : xbsIndex_r4/Slice  nbits=19  boolean_output=off  mode=Upper Bit Location + Width  bit1=-95  base1=MSB of Input  bit0=0  base0=LSB of Input  dbl_ovrd=off  block_type=slice
  slice4 : xbsIndex_r4/Slice  nbits=19  boolean_output=off  mode=Upper Bit Location + Width  bit1=-76  base1=MSB of Input  bit0=0  base0=LSB of Input  dbl_ovrd=off  block_type=slice
  slice5 : xbsIndex_r4/Slice  nbits=19  boolean_output=off  mode=Upper Bit Location + Width  bit1=-57  base1=MSB of Input  bit0=0  base0=LSB of Input  dbl_ovrd=off  block_type=slice
  slice6 : xbsIndex_r4/Slice  nbits=19  boolean_output=off  mode=Upper Bit Location + Width  bit1=-38  base1=MSB of Input  bit0=0  base0=LSB of Input  dbl_ovrd=off  block_type=slice
  slice7 : xbsIndex_r4/Slice  nbits=19  boolean_output=off  mode=Upper Bit Location + Width  bit1=-19  base1=MSB of Input  bit0=0  base0=LSB of Input  dbl_ovrd=off  block_type=slice
  slice8 : xbsIndex_r4/Slice  nbits=19  boolean_output=off  mode=Upper Bit Location + Width  bit1=0  base1=MSB of Input  bit0=0  base0=LSB of Input  dbl_ovrd=off  block_type=slice
  msb_out8 : Outport
  out7 : Outport  Port=2
  out6 : Outport  Port=3
  out5 : Outport  Port=4
  out4 : Outport  Port=5
  out3 : Outport  Port=6
  out2 : Outport  Port=7
  lsb_out1 : Outport  Port=8  VectorParamsAs1DForOutWhenUnconnected=off
  wires:
  reinterpret1/1 -> lsb_out1/1
  slice1/1 -> reinterpret1/1
  reinterpret2/1 -> out2/1
  slice2/1 -> reinterpret2/1
  reinterpret3/1 -> out3/1
  slice3/1 -> reinterpret3/1
  reinterpret4/1 -> out4/1
  slice4/1 -> reinterpret4/1
  reinterpret5/1 -> out5/1
  slice5/1 -> reinterpret5/1
  reinterpret6/1 -> out6/1
  slice6/1 -> reinterpret6/1
  reinterpret7/1 -> out7/1
  slice7/1 -> reinterpret7/1
  reinterpret8/1 -> msb_out8/1
  slice8/1 -> reinterpret8/1
  bus_in/1 -> slice1/1, slice2/1, slice3/1, slice4/1, slice5/1, slice6/1, slice7/1, slice8/1

== system rfsoc4x2_ospfb_128/fft_wideband_real1/fft_direct/butterfly1_0/bus_add/op_bussify ==
  in1 : Inport
  in2 : Inport  Port=2
  in3 : Inport  Port=3
  in4 : Inport  Port=4
  in5 : Inport  Port=5
  in6 : Inport  Port=6
  in7 : Inport  Port=7
  in8 : Inport  Port=8
  concatenate : xbsIndex_r4/Concat  num_inputs=8  dbl_ovrd=off  block_type=concat
  reinterpret{1..8} (8 alike) : xbsIndex_r4/Reinterpret  force_arith_type=on  arith_type=Unsigned  force_bin_pt=on  bin_pt=0  block_type=reinterpret
      reinterpret1 settings: infoedit="Changes signal type without altering the binary representation.   You can changed the signal between signed and unsigned, and relocate the binary point.<br><br>Hardware notes: In hardware this block costs nothing.<br><br>Example:  Suppose the input is 6 bits wide, signed, with 2 fractional bits, and the output is forced to unsigned with 0 fractional bits.  Then an input of -2.0 (1110.00 in binary 2's complement) becomes an output of 56 (111000 in binary)."
      reinterpret2 settings: infoedit="Changes signal type without altering the binary representation.   You can changed the signal between signed and unsigned, and relocate the binary point.<br><br>Hardware notes: In hardware this block costs nothing.<br><br>Example:  Suppose the input is 6 bits wide, signed, with 2 fractional bits, and the output is forced to unsigned with 0 fractional bits.  Then an input of -2.0 (1110.00 in binary 2's complement) becomes an output of 56 (111000 in binary)."
  bus_out : Outport  VectorParamsAs1DForOutWhenUnconnected=off
  wires:
  reinterpret8/1 -> concatenate/8
  in8/1 -> reinterpret8/1
  reinterpret7/1 -> concatenate/7
  in7/1 -> reinterpret7/1
  reinterpret6/1 -> concatenate/6
  in6/1 -> reinterpret6/1
  reinterpret5/1 -> concatenate/5
  in5/1 -> reinterpret5/1
  reinterpret4/1 -> concatenate/4
  in4/1 -> reinterpret4/1
  reinterpret3/1 -> concatenate/3
  in3/1 -> reinterpret3/1
  reinterpret2/1 -> concatenate/2
  in2/1 -> reinterpret2/1
  reinterpret1/1 -> concatenate/1
  in1/1 -> reinterpret1/1
  concatenate/1 -> bus_out/1

== system rfsoc4x2_ospfb_128/fft_wideband_real1/fft_direct/butterfly1_0/bus_convert/bussify ==
  in1 : Inport
  in2 : Inport  Port=2
  in3 : Inport  Port=3
  in4 : Inport  Port=4
  in5 : Inport  Port=5
  in6 : Inport  Port=6
  in7 : Inport  Port=7
  in8 : Inport  Port=8
  in9 : Inport  Port=9
  in10 : Inport  Port=10
  in11 : Inport  Port=11
  in12 : Inport  Port=12
  in13 : Inport  Port=13
  in14 : Inport  Port=14
  in15 : Inport  Port=15
  in16 : Inport  Port=16
  concatenate : xbsIndex_r4/Concat  num_inputs=16  dbl_ovrd=off  block_type=concat
  reinterpret{1..16} (16 alike) : xbsIndex_r4/Reinterpret  force_arith_type=on  arith_type=Unsigned  force_bin_pt=on  bin_pt=0  block_type=reinterpret
      reinterpret1 settings: infoedit="Changes signal type without altering the binary representation.   You can changed the signal between signed and unsigned, and relocate the binary point.<br><br>Hardware notes: In hardware this block costs nothing.<br><br>Example:  Suppose the input is 6 bits wide, signed, with 2 fractional bits, and the output is forced to unsigned with 0 fractional bits.  Then an input of -2.0 (1110.00 in binary 2's complement) becomes an output of 56 (111000 in binary)."
      reinterpret2 settings: infoedit="Changes signal type without altering the binary representation.   You can changed the signal between signed and unsigned, and relocate the binary point.<br><br>Hardware notes: In hardware this block costs nothing.<br><br>Example:  Suppose the input is 6 bits wide, signed, with 2 fractional bits, and the output is forced to unsigned with 0 fractional bits.  Then an input of -2.0 (1110.00 in binary 2's complement) becomes an output of 56 (111000 in binary)."
  bus_out : Outport  VectorParamsAs1DForOutWhenUnconnected=off
  wires:
  reinterpret16/1 -> concatenate/16
  in16/1 -> reinterpret16/1
  reinterpret15/1 -> concatenate/15
  in15/1 -> reinterpret15/1
  reinterpret14/1 -> concatenate/14
  in14/1 -> reinterpret14/1
  reinterpret13/1 -> concatenate/13
  in13/1 -> reinterpret13/1
  reinterpret12/1 -> concatenate/12
  in12/1 -> reinterpret12/1
  reinterpret11/1 -> concatenate/11
  in11/1 -> reinterpret11/1
  reinterpret10/1 -> concatenate/10
  in10/1 -> reinterpret10/1
  reinterpret9/1 -> concatenate/9
  in9/1 -> reinterpret9/1
  reinterpret8/1 -> concatenate/8
  in8/1 -> reinterpret8/1
  reinterpret7/1 -> concatenate/7
  in7/1 -> reinterpret7/1
  reinterpret6/1 -> concatenate/6
  in6/1 -> reinterpret6/1
  reinterpret5/1 -> concatenate/5
  in5/1 -> reinterpret5/1
  reinterpret4/1 -> concatenate/4
  in4/1 -> reinterpret4/1
  reinterpret3/1 -> concatenate/3
  in3/1 -> reinterpret3/1
  reinterpret2/1 -> concatenate/2
  in2/1 -> reinterpret2/1
  reinterpret1/1 -> concatenate/1
  in1/1 -> reinterpret1/1
  concatenate/1 -> bus_out/1
